simulink model "SinglePhaseGridSolarPV"  (R2025b)
settings: Solver=ode23t  StartTime=0.0  StopTime=simulation.timeSim  FixedStep=0.001  MaxStep=1/(5*solarPlant.switchFrequency)  RelTol=1e-3  AbsTol=1e-3  EnableMultiTasking=on
PreLoadFcn:
  | run('SinglePhaseGridSolarPVData');
undefined symbols (not defined in the file): closedLoop, controller, grid, protection, sensor, solarPanel, solarPlant
libraries: simulink x19, fl_lib x16, nesl_utility x16, ee_lib x8, mcbeeMathTransformLib x2, simulink_extras x1, eeSinusoidalMeasurement x1, eeRmsMeasurement x1, eePwmGenerator x1
(part 1 of 2)
CloseFcn:
  | try, close(figHandleGridconnectedSolarSinglePhase), end
  | try, clear figHandleGridconnectedSolarSinglePhase, end
  | 
  | clear simlog_SinglePhaseGridSolarPV
  | clear warnState
  | clear solarPanel grid solarPlant sensor controller protection simulation
  | clear inductorDesign closedLoop
  | clear remainingPowerPerString
  | clear simulation  MPPT  powerCircuit
  | clear incrementalConductance perturbationAndObservation
  | clear discrete average continuous
  | clear modelName X U idx t x y X U A B C D G closedLoop
  | clear npts f G magline_h phsline_h presentMPPTVariant presentInverterVariant
  | clear i inverter
  | clear xout yout tout
Description:
  | Single-Phase Grid-Connected Solar Photovoltaic System
  | 
  | %
settings Model: Creator=The MathWorks, Inc.
settings SolverCC: AlgebraicLoopSolver=TrustRegion
settings DataIOCC: MaxDataPoints=285000  SaveFormat=Array  SaveState=on  SignalLogging=off  DSMLogging=off  ReturnWorkspaceOutputs=off  SignalLoggingName=logsout_StepperMotorValidation
settings OptimizationCC: ReuseModelBlockBuffer=off  ExpressionDepthLimit=2147483647.0  InitFltsAndDblsToZero=on  LifeSpan=inf
settings DebuggingCC: UnderspecifiedInitializationDetection=Classic  MergeDetectMultiDrivingBlocksExec=none  FcnCallInpInsideContextMsg=warning  UnconnectedInputMsg=warning  UnconnectedOutputMsg=warning  UnconnectedLineMsg=warning  StateNameClashWarn=warning  PregeneratedLibrarySubsystemCodeDiagnostic=none  SFUnexpectedBacktrackingDiag=warning  SFNoUnconditionalDefaultTransitionDiag=warning  SFExecutionAtInitializationDiag=none  ArithmeticOperatorsInVariantConditions=warning
settings HardwareCC: ProdBitPerPointer=32.0  ProdBitPerSizeT=32.0  ProdBitPerPtrDiffT=32.0  ProdLargestAtomicFloat=None  ProdIntDivRoundTo=Undefined  ProdEndianess=Unspecified  ProdWordSize=32.0  ProdHWDeviceType=32-bit Generic
settings ModelReferenceCC: EnableRefExpFcnMdlSchedulingChecks=on  PropagateSignalLabelsOutOfModel=off
settings SFSimCC: SimUseLocalCustomCode=off
settings RTWCC: RTWUseLocalCustomCode=off  GPUComputeCapability=3.5  DLArmComputeVersion=19.05
settings CodeAppCC: StateflowObjectComments=on
settings GRTTargetCC: TargetLangStandard=C89/C90 (ANSI)  CombineOutputUpdateFcns=off  GRTInterface=on
settings ConfigComp: CovScope=ReferencedModels  CovMetricSettings=dw  CovSaveCumulativeToWorkspaceVar=on  CovSaveSingleToWorkspaceVar=on  CovExternalEMLEnable=off  CovSFcnEnable=off
settings SimscapeCC: SimscapeLogType=all  SimscapeLogSimulationStatistics=on  SimscapeLogName=simlog_SinglePhaseGridSolarPV  SimscapeLogLimitData=off  SimscapeLogDataHistory=285000.0

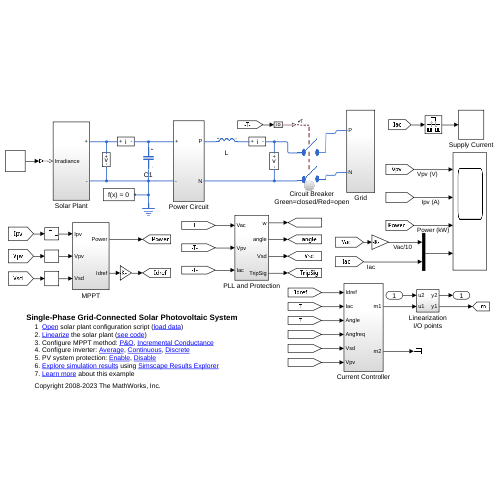
[thumbnail: Simulink's stored preview of the top-level diagram]
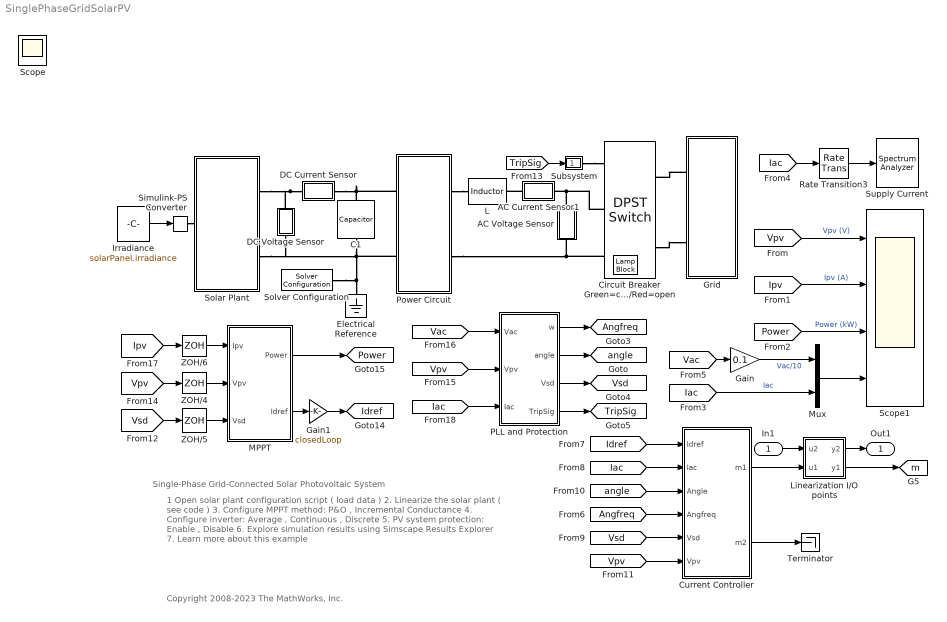
== system SinglePhaseGridSolarPV ==
  note: 1 Open solar plant configuration script ( load data )
      | 2. Linearize the solar plant ( see code )
      | 3. Configure MPPT method: P&O , Incremental Conductance
      | 4. Configure inverter: Average , Continuous , Discrete
      | 5. PV system protection: Enable , Disable
      | 6. Explore simulation results using Simscape Results Explorer
      | 7. Learn more about this example
  note: Single-Phase Grid-Connected Solar Photovoltaic System
  note: Copyright 2008-2023 The MathWorks, Inc.
  In1 : Inport
  " " : LampBlock  LabelPosition=Hide  DefaultColor=[192.0, 192.0, 192.0]
  AC Current Sensor1 : Subsystem
      mask Display: disp('i');
  AC Voltage Sensor : Subsystem
      mask Display: disp('v')
  C1 : fl_lib/Electrical/Electrical Elements/Capacitor  c=solarPlant.capacitance F  r=1e-6 Ohm  g=0 1/Ohm  i_specify=off  i_priority=High  i=0 A  i_nominal_specify=off  i_nominal_value=1  i_nominal_unit=A  v_specify=off  v_priority=High  v=0 V  v_nominal_specify=off  v_nominal_value=1  v_nominal_unit=V  vc_specify=on  vc_priority=High  vc=solarPlant.DCMPPTValue V  vc_nominal_specify=off  vc_nominal_value=1  vc_nominal_unit=V
  Circuit Breaker Green=closed/Red=open : ee_lib/Switches & Breakers/DPST Switch  R_closed=0.001 Ohm  G_open=1e-6 S  Threshold=0.5 V  Width=0 V  model_dynamics=0  t_on=1e-3 s  t_off=1e-3 s  initial_vT=0 V
      settings: InternalSimscapePortConfiguration="{\"Bottom\":[],\"Left\":[{\"id\":\"vT\",\"label\":\"vT\",\"type\":\"input\"},{\"id\":\"p1\",\"label\":\"\",\"type\":\"foundation.electrical.electrical\"},{\"id\":\"p2\",\"label\":\"\",\"type\":\"foundation.electrical.electrical\"}],\"Right\":[{\"id\":\"n1\",\"label\":\"\",\"type\":\"foundation.electrical.electrical\"},{\"id\":\"n2\",\"label\":\"\",\"type\":\"foundation.electrical.electrical\"}],\"Top\":[]}"
  Current Controller : Subsystem
  DC Current Sensor : Subsystem
      mask Display: disp('i')
  DC Voltage Sensor : Subsystem
      mask Display: disp('v');
  Electrical Reference : fl_lib/Electrical/Electrical Elements/Electrical Reference
  Gain : Gain  Gain=0.1
  Gain1 : Gain  Gain=closedLoop
  Grid : Subsystem
  Irradiance : Constant  Value=solarPanel.irradiance
  L : fl_lib/Electrical/Electrical Elements/Inductor  l=solarPlant.lineInductance H  r=solarPlant.inductorResistance Ohm  g=1e-9 1/Ohm  i_specify=off  i_priority=High  i=0 A  i_nominal_specify=off  i_nominal_value=1  i_nominal_unit=A  v_specify=off  v_priority=High  v=0 V  v_nominal_specify=off  v_nominal_value=1  v_nominal_unit=V  i_L_specify=on  i_L_priority=High  i_L=0 A  i_L_nominal_specify=off  i_L_nominal_value=1  i_L_nominal_unit=A
      settings: LogSimulationData=on
  Linearization I/O points : Subsystem
  MPPT : Subsystem
  Mux : Mux  Inputs=2
  PLL and Protection : Subsystem
  Power Circuit : Subsystem
  Rate Transition3 : RateTransition  OutPortSampleTime=1e-4
  Scope1 : Scope  NumInputPorts=4
      settings: TimeSpan=simulation.timeSim  ActiveDisplayYMinimum=-79.35501  ActiveDisplayYMaximum=714.19509
  Simulink-PS Converter : nesl_utility/Simulink-PS Converter  PhysicalDomain=network_engine_domain  SubClassName=ps_input  LeftPortType=input  RightPortType=output  PseudoPeriodic=off  Frequencies=[]  NoiseDistribution=none  NoiseParameters=[]  Unit=1  AffineConversion=off  FilteringAndDerivatives=provide  SimscapeFilterOrder=1  InputFilterTimeConstant=0.001  UdotUserProvided=0
  Solar Plant : Subsystem
  Solver Configuration : nesl_utility/Solver Configuration  PhysicalDomain=network_engine_domain  SubClassName=solver  LeftPortType=input  RightPortType=generic  Tones=[]  Harmonics=[]  SimulateNoise=off  Profile=off  UseLocalSampling=off  EnableSwitchedLinearOptims=on  FrequencyDomain=off  UseCCode=off  RelTol=0.001  AbsTol=1e-06  MinStep=1e-09  ToWorkspace=off  RevertToSquareIcSolve=off  NumHomotopyIterations=100  PhasorMode=off  PhasorModeNumHarmonics=1  ConsistencySolver=NEWTON_FTOL  IndexReductionMethod=DerivativeReplacement  DoDC=off  ResidualTolerance=1e-9  ConsistencyTolSource=GLOBAL  ConsistencyAbsTol=0.001  ConsistencyRelTol=0.001  ConsistencyTolFactor=0.001  UseLocalSolver=off  LocalSolverChoice=NE_TRAPEZOIDAL_ADVANCER  ResolveIndetEquations=on  FunctionEvalNumThread=1  LocalSolverSampleTime=1e-7  DoFixedCost=off  MaxNonlinIter=10  MaxModeIter=2  ComputeImpulses=off  ImpulseIterations=2  LinearAlgebra=auto  LinearAlgebraNumThread=0  EquationFormulation=NE_TIME_EF  DelaysMemoryBudget=1024  AutomaticFiltering=on  FilteringTimeConstant=0.001  PartitionStorageMethod=AS_NEEDED  PartitionMemoryBudget=1024  PartitionMethod=FAST  MultibodyUseLocalSolver=off  MultibodyLocalSolverChoice=ODE1  MultibodyLocalSolverSampleTime=0.001
  Subsystem : Subsystem
  Supply Current : SpectrumAnalyzer  WindowPosition=[886 344 803 532]  SpectrumType=RMS  Method=Welch  PlotAsTwoSidedSpectrum=off  FrequencyScale=Log  AxesScaling=Manual  RBWSource=Property  RBW=9  Span=5000  CenterFrequency=2500  StartFrequency=0  OverlapPercent=90  AveragingMethod=Running  SpectrumUnits=Vrms  YLimits=[-2.1499375144550283423,19.349555712689415543]  ColorLimits=[0.0061790664803535039207,16.888204283875005274]  AllowFFTLengthLessThanSamplesPerUpdate=on
      settings: OpenAtSimulationStart=off
  Terminator : Terminator
  ZOH/4 : ZeroOrderHold  SampleTime=solarPlant.timeMPPT
  ZOH/5 : ZeroOrderHold  SampleTime=solarPlant.timeMPPT
  ZOH/6 : ZeroOrderHold  SampleTime=solarPlant.timeMPPT
  Out1 : Outport  VectorParamsAs1DForOutWhenUnconnected=off
  Scope : Scope
      settings: ActiveDisplayYMinimum=-0.0002  ActiveDisplayYMaximum=0.0018
  tag scope: Angfreq=global, Idref=global, Power=global, TripSig=global, Vsd=global, angle=global, m=global
  wires:
  Mux/1 -> Scope1/4
  Irradiance/1 -> Simulink-PS Converter/1
  [Vsd] -> ZOH/5/1
  [Vpv] -> ZOH/4/1
  [Iac] -> Current Controller/2(Iac)
  Current Controller/1(m1) -> Linearization I/O points/2(u1)
  [Vac] -> Gain/1
  PLL and Protection/4(TripSig) -> [TripSig]
  Rate Transition3/1 -> Supply Current/1
  PLL and Protection/2(angle) -> [angle]
  [TripSig] -> Subsystem/1(i)
  Linearization I/O points/1(y2) -> Out1/1
  [Iac] -> PLL and Protection/3(Iac)
  ZOH/5/1 -> MPPT/3(Vsd)
  PLL and Protection/3(Vsd) -> [Vsd]
  [Vac] -> PLL and Protection/1(Vac)
  [Ipv] -> Scope1/2  "Ipv (A)"
  Linearization I/O points/2(y1) -> [m]
  [Vsd] -> Current Controller/5(Vsd)
  Current Controller/2(m2) -> Terminator/1
  PLL and Protection/1(w) -> [Angfreq]
  [Angfreq] -> Current Controller/4(Angfreq)
  [Ipv] -> ZOH/6/1
  [Vpv] -> Scope1/1  "Vpv (V)"
  [Idref] -> Current Controller/1(Idref)
  MPPT/2(Idref) -> Gain1/1
  Gain1/1 -> [Idref]
  [Vpv] -> PLL and Protection/2(Vpv)
  [Vpv] -> Current Controller/6(Vpv)
  In1/1 -> Linearization I/O points/1(u2)
  [Iac] -> Mux/2  "Iac"
  [Power] -> Scope1/3  "Power (kW)"
  [angle] -> Current Controller/3(Angle)
  ZOH/4/1 -> MPPT/2(Vpv)
  ZOH/6/1 -> MPPT/1(Ipv)
  Gain/1 -> Mux/1  "Vac/10"
  [Iac] -> Rate Transition3/1
  MPPT/1(Power) -> [Power]
  connections:
  Power Circuit/LConn2 -- Electrical Reference/LConn1 -- Solver Configuration/RConn1 -- C1/RConn1 -- Solar Plant/RConn2 -- DC Voltage Sensor/LConn1
  Circuit Breaker Green=closed/Red=open/LConn3 -- Power Circuit/RConn2 -- AC Voltage Sensor/LConn1
  DC Current Sensor/RConn1 -- Solar Plant/RConn1 -- DC Voltage Sensor/RConn1
  AC Current Sensor1/LConn1 -- AC Voltage Sensor/RConn1 -- Circuit Breaker Green=closed/Red=open/LConn2
  Power Circuit/LConn1 -- DC Current Sensor/LConn1 -- C1/LConn1
  Grid/LConn1 -- Circuit Breaker Green=closed/Red=open/RConn1
  Circuit Breaker Green=closed/Red=open/RConn2 -- Grid/LConn2
  AC Current Sensor1/RConn1 -- L/RConn1
  Subsystem/RConn1 -- Circuit Breaker Green=closed/Red=open/LConn1
  Simulink-PS Converter/RConn1 -- Solar Plant/LConn1
  Power Circuit/RConn1 -- L/LConn1

== system SinglePhaseGridSolarPV/AC Current Sensor1 ==
  Current Sensor : fl_lib/Electrical/Electrical Sensors/Current Sensor
  PS-Simulink Converter : nesl_utility/PS-Simulink Converter  PhysicalDomain=network_engine_domain  SubClassName=ps_output  LeftPortType=input  RightPortType=output  PseudoPeriodic=off  Frequencies=[]  VectorFormat=1-D array  Unit=1  AffineConversion=off
  Sensor dynamics : TransferFcn  Numerator=1  Denominator=[1/sensor.samplingFreq 1]
  - : PMIOPort  Side=Left
  + : PMIOPort  Port=2  Side=Right
  tag scope: Iac=global
  wires:
  PS-Simulink Converter/1 -> Sensor dynamics/1
  Sensor dynamics/1 -> [Iac]
  connections:
  Current Sensor/RConn1 -- PS-Simulink Converter/LConn1
  +/RConn1 -- Current Sensor/LConn1
  Current Sensor/RConn2 -- -/RConn1

== system SinglePhaseGridSolarPV/AC Voltage Sensor ==
  PS-Simulink Converter : nesl_utility/PS-Simulink Converter  PhysicalDomain=network_engine_domain  SubClassName=ps_output  LeftPortType=input  RightPortType=output  PseudoPeriodic=off  Frequencies=[]  VectorFormat=1-D array  Unit=1  AffineConversion=off
  Sensor dynamics : TransferFcn  Numerator=1  Denominator=[1/sensor.samplingFreq 1]
  Voltage Sensor : fl_lib/Electrical/Electrical Sensors/Voltage Sensor
  - : PMIOPort  Side=Left
  + : PMIOPort  Port=2  Side=Right
  tag scope: Vac=global
  wires:
  PS-Simulink Converter/1 -> Sensor dynamics/1
  Sensor dynamics/1 -> [Vac]
  connections:
  Voltage Sensor/RConn2 -- -/RConn1
  Voltage Sensor/RConn1 -- PS-Simulink Converter/LConn1
  Voltage Sensor/LConn1 -- +/RConn1

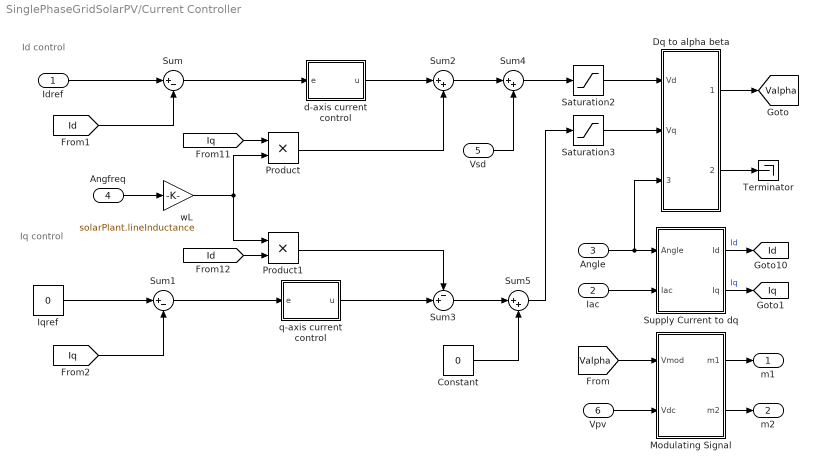
== system SinglePhaseGridSolarPV/Current Controller ==
  note: Iq control
  note: Id control
  Idref : Inport
  Iac : Inport  Port=2
  Angle : Inport  Port=3
  Angfreq : Inport  Port=4
  Vsd : Inport  Port=5
  Vpv : Inport  Port=6
  Constant : Constant  Value=0
  Dq to alpha beta : Subsystem
  Iqref : Constant  Value=0
  Modulating Signal : Subsystem
  Product : Product
  Product1 : Product
  Saturation2 : Saturate  UpperLimit=controller.currentVoltMax*1.5  LowerLimit=-1*controller.currentVoltMax*1.5
  Saturation3 : Saturate  UpperLimit=controller.currentVoltMax*1.5  LowerLimit=-1*controller.currentVoltMax*1.5
  Sum : Sum  Inputs=|+-
  Sum1 : Sum  Inputs=|+-
  Sum2 : Sum  Inputs=|++
  Sum3 : Sum  Inputs=-+|
  Sum4 : Sum  Inputs=|++
  Sum5 : Sum  Inputs=|++
  Supply Current to dq : Subsystem
  Terminator : Terminator
  d-axis current control : Subsystem
  q-axis current control : Subsystem
  wL : Gain  Gain=solarPlant.lineInductance
  m1 : Outport  VectorParamsAs1DForOutWhenUnconnected=off
  m2 : Outport  Port=2  VectorParamsAs1DForOutWhenUnconnected=off
  tag scope: Id=global, Iq=global, Valpha=global
  wires:
  Sum1/1 -> q-axis current control/1(e)
  wL/1 -> Product/2, Product1/1
  [Id] -> Product1/2
  [Iq] -> Product/1
  Product1/1 -> Sum3/1
  Product/1 -> Sum2/2
  Sum3/1 -> Sum5/1
  Sum2/1 -> Sum4/1
  Modulating Signal/1(m1) -> m1/1
  Modulating Signal/2(m2) -> m2/1
  Sum4/1 -> Saturation2/1
  Sum5/1 -> Saturation3/1
  Angfreq/1 -> wL/1
  Constant/1 -> Sum5/2
  Angle/1 -> Dq to alpha beta/3(angle), Supply Current to dq/1(Angle)
  [Valpha] -> Modulating Signal/1(Vmod)
  Vpv/1 -> Modulating Signal/2(Vdc)
  Sum/1 -> d-axis current control/1(e)
  [Id] -> Sum/2
  d-axis current control/1(u) -> Sum2/1
  q-axis current control/1(u) -> Sum3/2
  Supply Current to dq/1(Id) -> [Id]  "Id"
  Supply Current to dq/2(Iq) -> [Iq]  "Iq"
  Iac/1 -> Supply Current to dq/2(Iac)
  Saturation2/1 -> Dq to alpha beta/1("Vd ")
  Saturation3/1 -> Dq to alpha beta/2(Vq)
  Vsd/1 -> Sum4/2
  Dq to alpha beta/1(Valpha) -> [Valpha]
  Dq to alpha beta/2(Vbeta) -> Terminator/1
  Iqref/1 -> Sum1/1
  [Iq] -> Sum1/2
  Idref/1 -> Sum/1

== system SinglePhaseGridSolarPV/DC Current Sensor ==
  Current Sensor : fl_lib/Electrical/Electrical Sensors/Current Sensor
      settings: LogSimulationData=on
  PS-Simulink Converter : nesl_utility/PS-Simulink Converter  PhysicalDomain=network_engine_domain  SubClassName=ps_output  LeftPortType=input  RightPortType=output  PseudoPeriodic=off  Frequencies=[]  VectorFormat=1-D array  Unit=1  AffineConversion=off
  Sensor dynamics : TransferFcn  Numerator=1  Denominator=[1/sensor.samplingFreq 1]
  - : PMIOPort  Side=Left
  + : PMIOPort  Port=2  Side=Right
  tag scope: Ipv=global
  wires:
  PS-Simulink Converter/1 -> Sensor dynamics/1
  Sensor dynamics/1 -> [Ipv]
  connections:
  Current Sensor/RConn2 -- -/RConn1
  +/RConn1 -- Current Sensor/LConn1
  Current Sensor/RConn1 -- PS-Simulink Converter/LConn1

== system SinglePhaseGridSolarPV/DC Voltage Sensor ==
  PS-Simulink Converter : nesl_utility/PS-Simulink Converter  PhysicalDomain=network_engine_domain  SubClassName=ps_output  LeftPortType=input  RightPortType=output  PseudoPeriodic=off  Frequencies=[]  VectorFormat=1-D array  Unit=1  AffineConversion=off
  Sensor dynamics : TransferFcn  Numerator=1  Denominator=[1/sensor.samplingFreq 1]
  Voltage Sensor : fl_lib/Electrical/Electrical Sensors/Voltage Sensor
      settings: LogSimulationData=on
  - : PMIOPort  Side=Left
  + : PMIOPort  Port=2  Side=Right
  tag scope: Vpv=global
  wires:
  PS-Simulink Converter/1 -> Sensor dynamics/1
  Sensor dynamics/1 -> [Vpv]
  connections:
  Voltage Sensor/LConn1 -- +/RConn1
  Voltage Sensor/RConn1 -- PS-Simulink Converter/LConn1
  Voltage Sensor/RConn2 -- -/RConn1

== system SinglePhaseGridSolarPV/Grid ==
  Controlled Voltage Source : fl_lib/Electrical/Electrical Sources/Controlled Voltage Source
  Grid Supply : Sin  Amplitude=grid.actualVoltage*sqrt(2)  Frequency=grid.frequency*2*pi  SampleTime=0
  Product : Product
  Simulink-PS Converter : nesl_utility/Simulink-PS Converter  PhysicalDomain=network_engine_domain  SubClassName=ps_input  LeftPortType=input  RightPortType=output  PseudoPeriodic=off  Frequencies=[]  NoiseDistribution=none  NoiseParameters=[]  Unit=1  AffineConversion=off  FilteringAndDerivatives=provide  SimscapeFilterOrder=1  InputFilterTimeConstant=0.001  UdotUserProvided=0
  Voltage Distrubance : Step  Time=10  Before=1  After=1.05  SampleTime=0
  P : PMIOPort  Side=Left
  N : PMIOPort  Port=2  Side=Left
  wires:
  Grid Supply/1 -> Product/2
  Product/1 -> Simulink-PS Converter/1
  Voltage Distrubance/1 -> Product/1
  connections:
  P/RConn1 -- Controlled Voltage Source/LConn1
  N/RConn1 -- Controlled Voltage Source/RConn2
  Simulink-PS Converter/RConn1 -- Controlled Voltage Source/RConn1

== system SinglePhaseGridSolarPV/Linearization I//O points ==
  u2 : Inport
  u1 : Inport  Port=2
  "Set to 1 for closed-loop operation, and set to 0 when linearizing" : Gain  Gain=closedLoop  SaturateOnIntegerOverflow=on  OutDataTypeStr=Inherit: Same as input  ParamDataTypeStr=Inherit: Same as input
  Sum1 : Sum  Inputs=++|  InputSameDT=on  SaturateOnIntegerOverflow=on  OutDataTypeStr=Inherit: Same as first input
  y2 : Outport  VectorParamsAs1DForOutWhenUnconnected=off
  y1 : Outport  Port=2  VectorParamsAs1DForOutWhenUnconnected=off
  wires:
  Sum1/1 -> y1/1
  u2/1 -> Sum1/1
  "Set to 1 for closed-loop operation, and set to 0 when linearizing"/1 -> Sum1/2
  u1/1 -> y2/1, "Set to 1 for closed-loop operation, and set to 0 when linearizing"/1

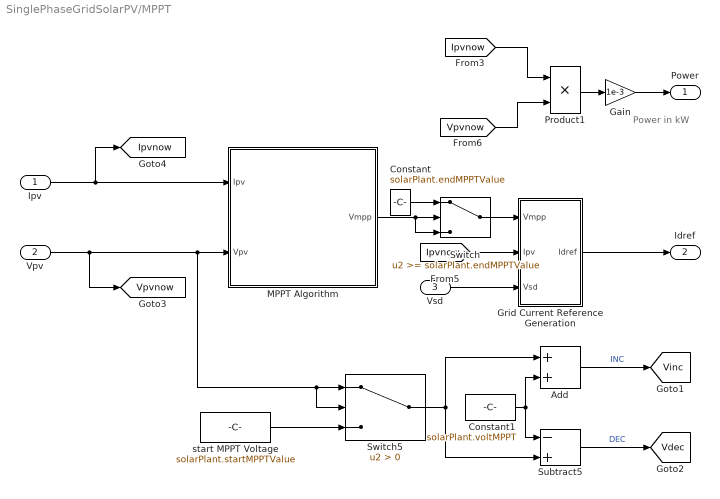
== system SinglePhaseGridSolarPV/MPPT ==
  note: Power in kW
  Ipv : Inport
  Vpv : Inport  Port=2
  Vsd : Inport  Port=3
  Add : Sum
  Constant : Constant  Value=solarPlant.endMPPTValue
  Constant1 : Constant  Value=solarPlant.voltMPPT
  Gain : Gain  Gain=1e-3
  Grid Current Reference Generation : Subsystem
  MPPT Algorithm : Subsystem  Variant=on
  Product1 : Product
  Subtract5 : Sum  Inputs=-+
  Switch : Switch  Threshold=solarPlant.endMPPTValue  SaturateOnIntegerOverflow=off  InputSameDT=off
  Switch5 : Switch  Criteria=u2 > Threshold  SaturateOnIntegerOverflow=off  InputSameDT=off
  start MPPT Voltage : Constant  Value=solarPlant.startMPPTValue
  Power : Outport  VectorParamsAs1DForOutWhenUnconnected=off
  Idref : Outport  Port=2  VectorParamsAs1DForOutWhenUnconnected=off
  tag scope: Ipvnow=global, Vdec=global, Vinc=global, Vpvnow=global
  wires:
  Switch5/1 -> Add/1, Subtract5/2
  Add/1 -> [Vinc]  "INC"
  start MPPT Voltage/1 -> Switch5/3
  Vpv/1 -> [Vpvnow], Switch5/2, Switch5/1, MPPT Algorithm/2(Vpv)
  Constant1/1 -> Add/2, Subtract5/1
  [Ipvnow] -> Grid Current Reference Generation/2(Ipv)
  Grid Current Reference Generation/1(Idref) -> Idref/1
  [Vpvnow] -> Product1/2
  [Ipvnow] -> Product1/1
  Product1/1 -> Gain/1
  Vsd/1 -> Grid Current Reference Generation/3(Vsd)
  Subtract5/1 -> [Vdec]  "DEC"
  Ipv/1 -> [Ipvnow], MPPT Algorithm/1(Ipv)
  Gain/1 -> Power/1
  Switch/1 -> Grid Current Reference Generation/1(Vmpp)
  MPPT Algorithm/1(Vmpp) -> Switch/3, Switch/2
  Constant/1 -> Switch/1

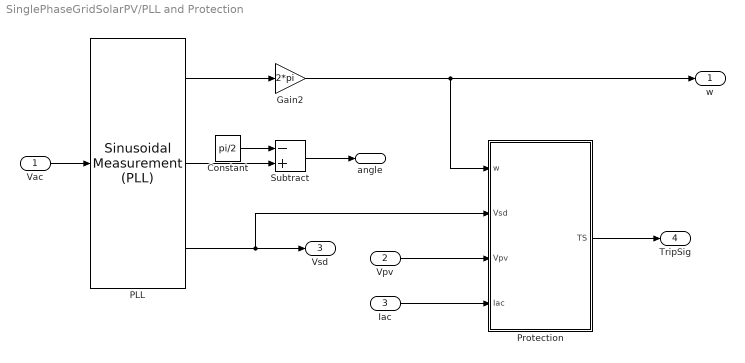
== system SinglePhaseGridSolarPV/PLL and Protection ==
  Vac : Inport
  Vpv : Inport  Port=2
  Iac : Inport  Port=3
  Constant : Constant  Value=pi/2
  Gain2 : Gain  Gain=2*pi
  PLL : eeSinusoidalMeasurement/Sinusoidal Measurement (PLL)  Ki_PD=600  Kp_LF=10  Ki_LF=200  F0=grid.frequency  Theta0=0  Mag0=grid.actualVoltage*sqrt(2)  Ts=0
  Protection : Subsystem
  Subtract : Sum  Inputs=-+
  w : Outport  VectorParamsAs1DForOutWhenUnconnected=off
  angle : Outport  Port=2  VectorParamsAs1DForOutWhenUnconnected=off
  Vsd : Outport  Port=3  VectorParamsAs1DForOutWhenUnconnected=off
  TripSig : Outport  Port=4  VectorParamsAs1DForOutWhenUnconnected=off
  wires:
  PLL/3 -> Vsd/1, Protection/2(Vsd)
  Gain2/1 -> Protection/1(w), w/1
  PLL/1 -> Gain2/1
  Vac/1 -> PLL/1
  Protection/1(TS) -> TripSig/1
  Vpv/1 -> Protection/3(Vpv)
  Iac/1 -> Protection/4(Iac)
  Subtract/1 -> angle/1
  PLL/2 -> Subtract/2
  Constant/1 -> Subtract/1

== system SinglePhaseGridSolarPV/Power Circuit ==
  Power Circuit : Subsystem  Variant=on  VariantControl=Variant1
  + : PMIOPort  Side=Left
  P : PMIOPort  Port=2  Side=Right
  N : PMIOPort  Port=3  Side=Right
  - : PMIOPort  Port=4  Side=Left
  wires:
  [m] -> Power Circuit/1(m)
  [TripSig] -> Power Circuit/2(TripSig)
  connections:
  +/RConn1 -- Power Circuit/LConn1
  -/RConn1 -- Power Circuit/LConn2
  P/RConn1 -- Power Circuit/RConn1
  N/RConn1 -- Power Circuit/RConn2

== system SinglePhaseGridSolarPV/Solar Plant ==
  Current-Controlled Current Source- Scale panel current to Np parallel strings : fl_lib/Electrical/Electrical Sources/Current-Controlled Current Source  K=-1*(solarPlant.numParallelPanel-1)  i1_specify=off  i1_priority=None  i1=0 A  i1_nominal_specify=off  i1_nominal_value=1  i1_nominal_unit=A  i2_specify=off  i2_priority=None  i2=0 A  i2_nominal_specify=off  i2_nominal_value=1  i2_nominal_unit=A
      settings: InternalSimscapePortConfiguration="{\"Bottom\":[],\"Left\":[{\"id\":\"p1\",\"label\":\"+\",\"type\":\"foundation.electrical.electrical\"},{\"id\":\"head\",\"label\":\"\",\"type\":\"foundation.electrical.electrical\"}],\"Right\":[{\"id\":\"n1\",\"label\":\"-\",\"type\":\"foundation.electrical.electrical\"},{\"id\":\"tail\",\"label\":\"\",\"type\":\"foundation.electrical.electrical\"}],\"Top\":[]}"
  Solar Panel : Subsystem  mask(Solar Panel){}
      mask help: Models a solar panel using a parallel-connected sting of solar cells. The solar cell strings are modeled using a single Solar Cell block from the Simscape(TM) Electrical(TM) Sources library.
      mask Display: image('SolarPanelValidationIcon.jpg')
  Voltage-Controlled Voltage Source - Scale panel voltage to Ns series panel : fl_lib/Electrical/Electrical Sources/Voltage-Controlled Voltage Source  K=-1*(solarPlant.numSeriesPanel-1)  v1_specify=off  v1_priority=None  v1=0 V  v1_nominal_specify=off  v1_nominal_value=1  v1_nominal_unit=V  v2_specify=off  v2_priority=None  v2=0 V  v2_nominal_specify=off  v2_nominal_value=1  v2_nominal_unit=V
      settings: InternalSimscapePortConfiguration="{\"Bottom\":[],\"Left\":[{\"id\":\"p1\",\"label\":\"+\",\"type\":\"foundation.electrical.electrical\"},{\"id\":\"p2\",\"label\":\"+\",\"type\":\"foundation.electrical.electrical\"}],\"Right\":[{\"id\":\"n1\",\"label\":\"-\",\"type\":\"foundation.electrical.electrical\"},{\"id\":\"n2\",\"label\":\"-\",\"type\":\"foundation.electrical.electrical\"}],\"Top\":[]}"
  + : PMIOPort  Side=Right
  Irradiance : PMIOPort  Port=2  Side=Left
  - : PMIOPort  Port=3  Side=Right
  connections:
  Voltage-Controlled Voltage Source - Scale panel voltage to Ns series panel/RConn2 -- Voltage-Controlled Voltage Source - Scale panel voltage to Ns series panel/RConn1 -- Solar Panel/RConn1
  Voltage-Controlled Voltage Source - Scale panel voltage to Ns series panel/LConn1 -- Current-Controlled Current Source- Scale panel current to Np parallel strings/LConn2 -- -/RConn1 -- Solar Panel/RConn2
  Current-Controlled Current Source- Scale panel current to Np parallel strings/RConn1 -- Current-Controlled Current Source- Scale panel current to Np parallel strings/RConn2 -- +/RConn1
  Current-Controlled Current Source- Scale panel current to Np parallel strings/LConn1 -- Voltage-Controlled Voltage Source - Scale panel voltage to Ns series panel/LConn2
  Solar Panel/LConn1 -- Irradiance/RConn1

== system SinglePhaseGridSolarPV/Subsystem ==
  i : Inport
  Data Type Conversion : DataTypeConversion  SaturateOnIntegerOverflow=off  RndMeth=Floor
  NOT : Logic  Operator=NOT  IconShape=distinctive  AllPortsSameDT=off  OutDataTypeStr=boolean
  Simulink-PS Converter : nesl_utility/Simulink-PS Converter  PhysicalDomain=network_engine_domain  SubClassName=ps_input  LeftPortType=input  RightPortType=output  PseudoPeriodic=off  Frequencies=[]  NoiseDistribution=none  NoiseParameters=[]  Unit=1  AffineConversion=off  FilteringAndDerivatives=provide  SimscapeFilterOrder=1  InputFilterTimeConstant=0.001  UdotUserProvided=0
  o : PMIOPort  Side=Right
  wires:
  NOT/1 -> Data Type Conversion/1
  i/1 -> NOT/1
  Data Type Conversion/1 -> Simulink-PS Converter/1
  connections:
  Simulink-PS Converter/RConn1 -- o/RConn1

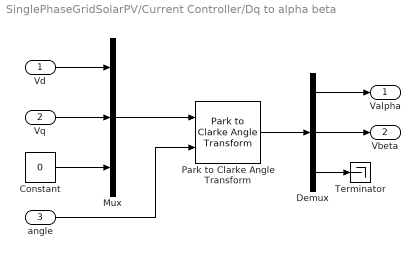
== system SinglePhaseGridSolarPV/Current Controller/Dq to alpha beta ==
  "Vd " : Inport
  Vq : Inport  Port=2
  angle : Inport  Port=3
  Constant : Constant  Value=0
  Demux : Demux  Outputs=3
  Mux : Mux  Inputs=3
  Park to Clarke Angle Transform : mcbeeMathTransformLib/Park to Clarke Angle Transform  AxisAlignment=D-axis  UseWithEmbedded=off  PhaseInput=Two inputs  ThetaInput=Sine and Cosine electrical position  AngleInput=Per-unit  N_points=1024
      settings: LibrarySourceBlock=|
      | eeTransforms/Park to Clarke
      | Angle Transform
  Terminator : Terminator
  Valpha : Outport  VectorParamsAs1DForOutWhenUnconnected=off
  Vbeta : Outport  Port=2  VectorParamsAs1DForOutWhenUnconnected=off
  wires:
  "Vd "/1 -> Mux/1
  Vq/1 -> Mux/2
  Constant/1 -> Mux/3
  Mux/1 -> Park to Clarke Angle Transform/1
  angle/1 -> Park to Clarke Angle Transform/2
  Park to Clarke Angle Transform/1 -> Demux/1
  Demux/1 -> Valpha/1
  Demux/2 -> Vbeta/1
  Demux/3 -> Terminator/1

== system SinglePhaseGridSolarPV/Current Controller/Modulating Signal ==
  Vmod : Inport
  Vdc : Inport  Port=2
  Gain : Gain  Gain=-1
  Normalize by DC voltage and disable if DC volts too low : Subsystem
  "[-1,1]" : Saturate  UpperLimit=1  LowerLimit=-1
  m1 : Outport  VectorParamsAs1DForOutWhenUnconnected=off
  m2 : Outport  Port=2  VectorParamsAs1DForOutWhenUnconnected=off
  wires:
  Normalize by DC voltage and disable if DC volts too low/1(y) -> "[-1,1]"/1
  Vdc/1 -> Normalize by DC voltage and disable if DC volts too low/2(v_dc)
  Vmod/1 -> Normalize by DC voltage and disable if DC volts too low/1(u)
  "[-1,1]"/1 -> m1/1, Gain/1
  Gain/1 -> m2/1

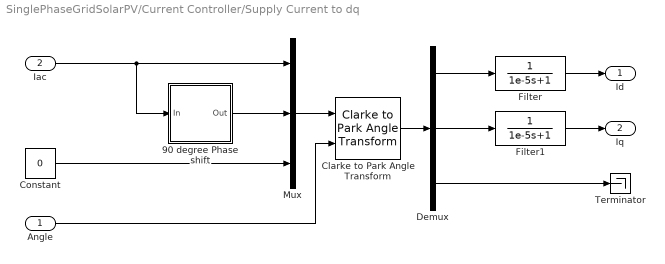
== system SinglePhaseGridSolarPV/Current Controller/Supply Current to dq ==
  Angle : Inport
  Iac : Inport  Port=2
  90 degree Phase shift : Subsystem
  Clarke to Park Angle Transform : mcbeeMathTransformLib/Clarke to Park Angle Transform  AxisAlignment=D-axis  UseWithEmbedded=off  PhaseInput=Two inputs  ThetaInput=Sine and Cosine electrical position  AngleInput=Per-unit  N_points=1024
      settings: LibrarySourceBlock=|
      | eeTransforms/Clarke to Park
      | Angle Transform
  Constant : Constant  Value=0
  Demux : Demux  Outputs=3
  Filter : TransferFcn  Denominator=[1e-5 1]
  Filter1 : TransferFcn  Denominator=[1e-5 1]
  Mux : Mux  Inputs=3
  Terminator : Terminator
  Id : Outport  VectorParamsAs1DForOutWhenUnconnected=off
  Iq : Outport  Port=2  VectorParamsAs1DForOutWhenUnconnected=off
  wires:
  Constant/1 -> Mux/3
  Mux/1 -> Clarke to Park Angle Transform/1
  Angle/1 -> Clarke to Park Angle Transform/2
  Demux/1 -> Filter/1
  Clarke to Park Angle Transform/1 -> Demux/1
  Demux/3 -> Terminator/1
  Filter/1 -> Id/1
  Iac/1 -> 90 degree Phase shift/1(In), Mux/1
  90 degree Phase shift/1(Out) -> Mux/2
  Filter1/1 -> Iq/1
  Demux/2 -> Filter1/1

== system SinglePhaseGridSolarPV/Current Controller/d-axis current control ==
  e : Inport
  Integrator : Integrator  LimitOutput=on  UpperSaturationLimit=controller.currentVoltMax  LowerSaturationLimit=-controller.currentVoltMax
  Ki : Gain  Gain=1/controller.currentPole
  Kp : Gain  Gain=controller.currentGain
  Saturation : Saturate  UpperLimit=controller.currentVoltMax  LowerLimit=-1*controller.currentVoltMax
  Sum7 : Sum  Inputs=|++
  u : Outport  VectorParamsAs1DForOutWhenUnconnected=off
  wires:
  Integrator/1 -> Sum7/2
  Saturation/1 -> u/1
  Sum7/1 -> Saturation/1
  e/1 -> Kp/1
  Kp/1 -> Ki/1, Sum7/1
  Ki/1 -> Integrator/1

== system SinglePhaseGridSolarPV/Current Controller/q-axis current control ==
  e : Inport
  Integrator : Integrator  LimitOutput=on  UpperSaturationLimit=controller.currentVoltMax  LowerSaturationLimit=-controller.currentVoltMax
  Ki : Gain  Gain=1/controller.currentPole
  Kp : Gain  Gain=controller.currentGain
  Saturation : Saturate  UpperLimit=controller.currentVoltMax  LowerLimit=-1*controller.currentVoltMax
  Sum7 : Sum  Inputs=|++
  u : Outport  VectorParamsAs1DForOutWhenUnconnected=off
  wires:
  Ki/1 -> Integrator/1
  Kp/1 -> Sum7/1, Ki/1
  e/1 -> Kp/1
  Sum7/1 -> Saturation/1
  Saturation/1 -> u/1
  Integrator/1 -> Sum7/2

== system SinglePhaseGridSolarPV/MPPT/Grid Current Reference Generation ==
  Vmpp : Inport
  Ipv : Inport  Port=2
  Vsd : Inport  Port=3
  Divide : Product  Inputs=*/
  Gain : Gain  Gain=2
  Product : Product
  Switch1 : Switch  Criteria=u2 > Threshold  Threshold=sqrt(2)*grid.actualVoltage*0.5  SaturateOnIntegerOverflow=off  InputSameDT=off
  Transfer Fcn (with initial outputs) : simulink_extras/Additional Linear/Transfer Fcn (with initial outputs)  N=[1]  D="[solarPlant.timeMPPT*70  1]"  Y0=solarPlant.initialIsdCurrent  U0=solarPlant.initialIsdCurrent
  Vsd Default : Constant  Value=sqrt(2)*grid.actualVoltage
  Idref : Outport  VectorParamsAs1DForOutWhenUnconnected=off
  wires:
  Divide/1 -> Gain/1
  Product/1 -> Divide/1
  Switch1/1 -> Divide/2
  Gain/1 -> Transfer Fcn (with initial outputs)/1
  Vmpp/1 -> Product/1
  Vsd/1 -> Switch1/2, Switch1/1
  Vsd Default/1 -> Switch1/3
  Ipv/1 -> Product/2
  Transfer Fcn (with initial outputs)/1 -> Idref/1

== system SinglePhaseGridSolarPV/MPPT/MPPT Algorithm ==
  Ipv : Inport
  Vpv : Inport  Port=2
  IncrementalConductance : Subsystem  VariantControl=incrementalConductance
  PerturbationAndObsrvation : Subsystem  VariantControl=perturbationAndObservation
  Vmpp : Outport  VectorParamsAs1DForOutWhenUnconnected=off

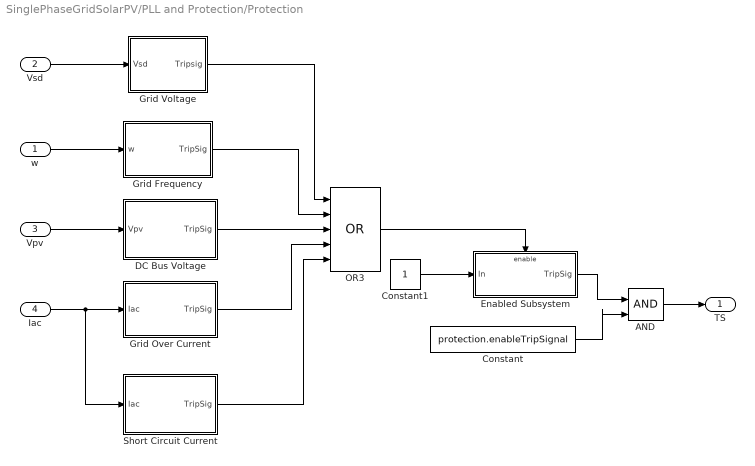
== system SinglePhaseGridSolarPV/PLL and Protection/Protection ==
  w : Inport
  Vsd : Inport  Port=2
  Vpv : Inport  Port=3
  Iac : Inport  Port=4
  AND : Logic  IconShape=distinctive  AllPortsSameDT=off  OutDataTypeStr=boolean
  Constant : Constant  Value=protection.enableTripSignal
  Constant1 : Constant
  DC Bus Voltage : Subsystem
  Enabled Subsystem : Subsystem  TreatAsAtomicUnit=on
  Grid Frequency : Subsystem
  Grid Over Current : Subsystem
  Grid Voltage : Subsystem
  OR3 : Logic  Operator=OR  Inputs=5  IconShape=distinctive  AllPortsSameDT=off  OutDataTypeStr=boolean
  Short Circuit Current : Subsystem
  TS : Outport  VectorParamsAs1DForOutWhenUnconnected=off
  wires:
  Constant1/1 -> Enabled Subsystem/1(In)
  Iac/1 -> Grid Over Current/1(Iac), Short Circuit Current/1(Iac)
  OR3/1 -> Enabled Subsystem/Enable
  Vsd/1 -> Grid Voltage/1(Vsd)
  Grid Voltage/1(Tripsig) -> OR3/1
  w/1 -> Grid Frequency/1(w)
  Grid Frequency/1(TripSig) -> OR3/2
  Vpv/1 -> DC Bus Voltage/1(Vpv)
  DC Bus Voltage/1(TripSig) -> OR3/3
  Grid Over Current/1(TripSig) -> OR3/4
  Short Circuit Current/1(TripSig) -> OR3/5
  Enabled Subsystem/1(TripSig) -> AND/1
  Constant/1 -> AND/2
  AND/1 -> TS/1

== system SinglePhaseGridSolarPV/Power Circuit/Power Circuit ==
  m : Inport
  TripSig : Inport  Port=2
  Average : Subsystem  VariantControl=average
  Continuous : Subsystem  VariantControl=continuous
  Discrete : Subsystem  VariantControl=discrete
  P : PMIOPort  Side=Right
  + : PMIOPort  Port=2  Side=Left
  - : PMIOPort  Port=3  Side=Left
  N : PMIOPort  Port=4  Side=Right

== system SinglePhaseGridSolarPV/Solar Plant/Solar Panel ==
  Current-Controlled Current Source : fl_lib/Electrical/Electrical Sources/Current-Controlled Current Source  K=-1*(solarPanel.numParallelCell-1)  i1_specify=off  i1_priority=None  i1=0 A  i1_nominal_specify=off  i1_nominal_value=1  i1_nominal_unit=A  i2_specify=off  i2_priority=None  i2=0 A  i2_nominal_specify=off  i2_nominal_value=1  i2_nominal_unit=A
      settings: InternalSimscapePortConfiguration="{\"Bottom\":[],\"Left\":[{\"id\":\"p1\",\"label\":\"+\",\"type\":\"foundation.electrical.electrical\"},{\"id\":\"head\",\"label\":\"\",\"type\":\"foundation.electrical.electrical\"}],\"Right\":[{\"id\":\"n1\",\"label\":\"-\",\"type\":\"foundation.electrical.electrical\"},{\"id\":\"tail\",\"label\":\"\",\"type\":\"foundation.electrical.electrical\"}],\"Top\":[]}"
  Solar Cell : ee_lib/Sources/Solar Cell  prm=1  Isc=solarPanel.shortCircuitCurrentPV/solarPanel.numParallelCell A  Voc=solarPanel.openCircuitVoltagePV/solarPanel.numSeriesCell V  Is=1e-6 A  Is2=0 A  Iph=7.34 A  Ir0=solarPanel.irradianceMeasurement W/m^2  ec=solarPanel.qualityFactor  N2=2  Rs=solarPanel.seriesResistance Ohm  Rp=inf Ohm  N_series=solarPanel.numSeriesCell-1  N_parallel=1  TIPH1=solarPanel.currentTemperatureCoeff 1/K  EG=1.11 eV  TXIS1=solarPanel.temperatureExponent  TXIS2=3  TRS1=0  TRP1=0  Tmeas=solarPanel.temperatureMeasurement degC  TFIXED=solarPanel.temperature degC  thermal_mass=100 J/K  initial_temperature=25 degC
  Ir : PMIOPort  Side=Left
  + : PMIOPort  Port=2  Side=Right
  - : PMIOPort  Port=3  Side=Right
  connections:
  Current-Controlled Current Source/LConn2 -- -/RConn1 -- Solar Cell/RConn1
  Ir/RConn1 -- Solar Cell/LConn1
  Current-Controlled Current Source/LConn1 -- Solar Cell/LConn2
  Current-Controlled Current Source/RConn1 -- Current-Controlled Current Source/RConn2 -- +/RConn1

== system SinglePhaseGridSolarPV/Current Controller/Modulating Signal/Normalize by DC voltage and disable if DC volts too low ==
  u : Inport
  v_dc : Inport  Port=2
  Min DC voltage : Constant  Value=0.5*solarPlant.startMPPTValue
  Product1 : Product  Inputs=*/  InputSameDT=on  SaturateOnIntegerOverflow=on  OutDataTypeStr=Inherit: Same as first input
  Switch1 : Switch  Threshold=0.5*solarPlant.maxPowerVoltage  SaturateOnIntegerOverflow=off
  y : Outport  VectorParamsAs1DForOutWhenUnconnected=off
  wires:
  Min DC voltage/1 -> Switch1/3
  Switch1/1 -> Product1/2
  v_dc/1 -> Switch1/2, Switch1/1
  u/1 -> Product1/1
  Product1/1 -> y/1

== system SinglePhaseGridSolarPV/Current Controller/Supply Current to dq/90 degree Phase shift ==
  In : Inport
  Gain : Gain  Gain=2
  Transfer Fcn : TransferFcn  Denominator=[1/(2*pi*grid.frequency) 1]
  Transfer Fcn1 : TransferFcn  Denominator=[1/(2*pi*grid.frequency) 1]
  Out : Outport  VectorParamsAs1DForOutWhenUnconnected=off
  wires:
  Transfer Fcn1/1 -> Gain/1
  Gain/1 -> Out/1
  Transfer Fcn/1 -> Transfer Fcn1/1
  In/1 -> Transfer Fcn/1

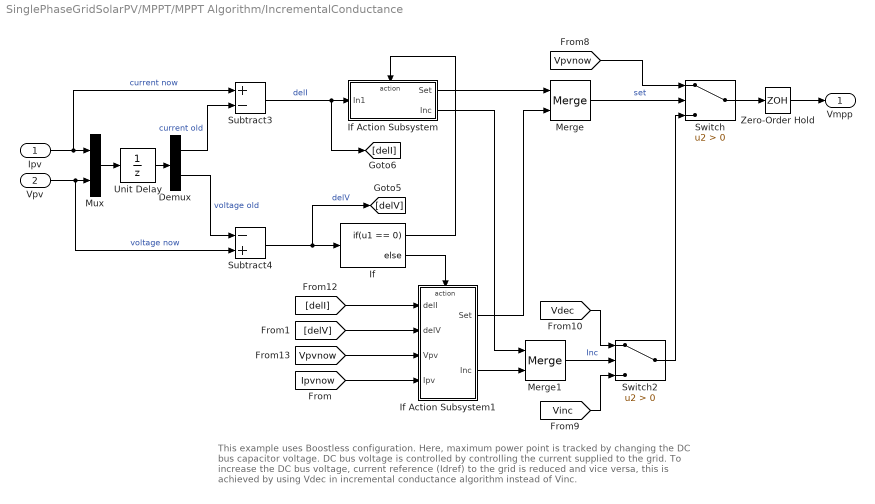
== system SinglePhaseGridSolarPV/MPPT/MPPT Algorithm/IncrementalConductance ==
  note: This example uses Boostless configuration. Here,  maximum power point is tracked by changing the DC bus capacitor voltage. DC bus voltage is controlled by controlling the current supplied to the grid.  To increase the DC bus voltage, current reference (Idref) to the grid is reduced and vice versa,
      | this is achieved by using Vdec in incremental conductance algorithm instead of Vinc.
  Ipv : Inport
  Vpv : Inport  Port=2
  Demux : Demux  Outputs=2
  If : If  IfExpression=u1 == 0
  If Action Subsystem : Subsystem  TreatAsAtomicUnit=on
  If Action Subsystem1 : Subsystem  TreatAsAtomicUnit=on
  Merge : Merge
  Merge1 : Merge
  Mux : Mux  Inputs=2
  Subtract3 : Sum  Inputs=+-
  Subtract4 : Sum  Inputs=-+
  Switch : Switch  Criteria=u2 > Threshold  SaturateOnIntegerOverflow=off  InputSameDT=off
  Switch2 : Switch  Criteria=u2 > Threshold  SaturateOnIntegerOverflow=off  InputSameDT=off
  Unit Delay : UnitDelay  InitialCondition=solarPlant.startMPPTValue  SampleTime=solarPlant.timeMPPT  HasFrameUpgradeWarning=on
  Zero-Order Hold : ZeroOrderHold  SampleTime=solarPlant.timeMPPT
  Vmpp : Outport  VectorParamsAs1DForOutWhenUnconnected=off
  wires:
  Merge1/1 -> Switch2/2  "Inc"
  [Vpvnow] -> Switch/1
  If Action Subsystem1/2(Inc) -> Merge1/2
  If Action Subsystem/2(Inc) -> Merge1/1
  If/2 -> If Action Subsystem1/Action
  If Action Subsystem/1(Set) -> Merge/1
  [delV] -> If Action Subsystem1/2(delV)
  [delI] -> If Action Subsystem1/1(delI)
  Merge/1 -> Switch/2  "set"
  If Action Subsystem1/1(Set) -> Merge/2
  If/1 -> If Action Subsystem/Action
  [Vpvnow] -> If Action Subsystem1/3(Vpv)
  Switch2/1 -> Switch/3
  [Ipvnow] -> If Action Subsystem1/4(Ipv)
  Ipv/1 -> Mux/1, Subtract3/1  "current now"
  Unit Delay/1 -> Demux/1
  Mux/1 -> Unit Delay/1
  Vpv/1 -> Subtract4/2, Mux/2  "voltage now"
  Demux/2 -> Subtract4/1  "voltage old"
  Demux/1 -> Subtract3/2  "current old"
  Subtract3/1 -> [delI], If Action Subsystem/1(In1)  "delI"
  Subtract4/1 -> [delV], If/1  "delV"
  [Vdec] -> Switch2/1
  [Vinc] -> Switch2/3
  Switch/1 -> Zero-Order Hold/1
  Zero-Order Hold/1 -> Vmpp/1

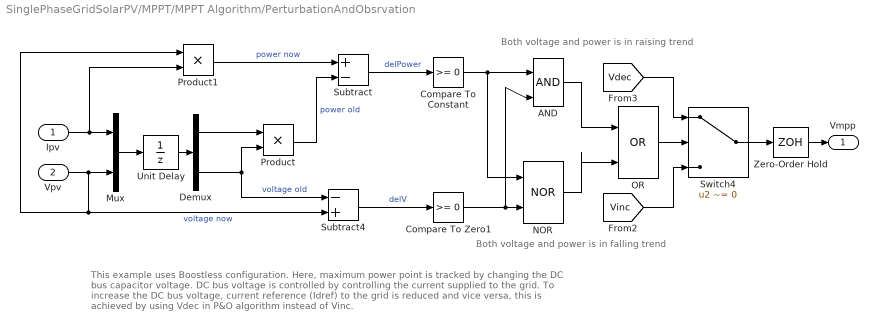
== system SinglePhaseGridSolarPV/MPPT/MPPT Algorithm/PerturbationAndObsrvation ==
  note: Both voltage and power is in falling trend
  note: Both voltage and power is in raising trend
  note: This example uses Boostless configuration. Here,  maximum power point is tracked by changing the DC bus capacitor voltage. DC bus voltage is controlled by controlling the current supplied to the grid.  To increase the DC bus voltage, current reference (Idref) to the grid is reduced and vice versa,
      | this is achieved by using Vdec in P&O algorithm instead of Vinc.
  Ipv : Inport
  Vpv : Inport  Port=2
  AND : Logic  IconShape=distinctive  AllPortsSameDT=off  OutDataTypeStr=boolean
  Compare To Constant : simulink/Logic and Bit Operations/Compare To Constant  relop=>=  const=0  OutDataTypeStr=boolean
  Compare To Zero1 : simulink/Logic and Bit Operations/Compare To Zero  relop=>=  OutDataTypeStr=boolean
  Demux : Demux  Outputs=2
  Mux : Mux  Inputs=2
  NOR : Logic  Operator=NOR  IconShape=distinctive  AllPortsSameDT=off  OutDataTypeStr=boolean
  OR : Logic  Operator=OR  IconShape=distinctive  AllPortsSameDT=off  OutDataTypeStr=boolean
  Product : Product
  Product1 : Product
  Subtract : Sum  Inputs=+-
  Subtract4 : Sum  Inputs=-+
  Switch4 : Switch  Criteria=u2 ~= 0  SaturateOnIntegerOverflow=off  InputSameDT=off
  Unit Delay : UnitDelay  InitialCondition=solarPlant.startMPPTValue  SampleTime=solarPlant.timeMPPT  HasFrameUpgradeWarning=on
  Zero-Order Hold : ZeroOrderHold  SampleTime=solarPlant.timeMPPT
  Vmpp : Outport  VectorParamsAs1DForOutWhenUnconnected=off
  wires:
  NOR/1 -> OR/2
  OR/1 -> Switch4/2
  Compare To Zero1/1 -> AND/2, NOR/2
  AND/1 -> OR/1
  Compare To Constant/1 -> AND/1, NOR/1
  Mux/1 -> Unit Delay/1
  Ipv/1 -> Product1/2, Mux/1
  Demux/1 -> Product/1
  Unit Delay/1 -> Demux/1
  Demux/2 -> Product/2, Subtract4/1  "voltage old"
  Vpv/1 -> Subtract4/2, Product1/1, Mux/2  "voltage now"
  Product1/1 -> Subtract/1  "power now"
  Product/1 -> Subtract/2  "power old"
  Subtract4/1 -> Compare To Zero1/1  "delV"
  Subtract/1 -> Compare To Constant/1  "delPower"
  Switch4/1 -> Zero-Order Hold/1
  Zero-Order Hold/1 -> Vmpp/1
  [Vinc] -> Switch4/3
  [Vdec] -> Switch4/1

== system SinglePhaseGridSolarPV/PLL and Protection/Protection/DC Bus Voltage ==
  Vpv : Inport
  Compare To Constant5 : simulink/Logic and Bit Operations/Compare To Constant  relop=>  const=protection.dcBusVoltageTripTime  OutDataTypeStr=boolean
  Compare To Constant6 : simulink/Logic and Bit Operations/Compare To Constant  relop=>  const=protection.dcBusMaxVoltage  OutDataTypeStr=boolean
  Compare To Constant7 : simulink/Logic and Bit Operations/Compare To Constant  relop=<  const=protection.dcBusMinVoltage  OutDataTypeStr=boolean
  Data Type Conversion1 : DataTypeConversion  SaturateOnIntegerOverflow=off  RndMeth=Floor
  Integrator1 : Integrator  ExternalReset=falling
  OR2 : Logic  Operator=OR  IconShape=distinctive  AllPortsSameDT=off  OutDataTypeStr=boolean
  Transfer Fcn2 : TransferFcn  Denominator=[1e-4 1]
  TripSig : Outport  VectorParamsAs1DForOutWhenUnconnected=off
  wires:
  Compare To Constant6/1 -> OR2/2
  Transfer Fcn2/1 -> Compare To Constant6/1, Compare To Constant7/1
  Compare To Constant7/1 -> OR2/1
  Vpv/1 -> Transfer Fcn2/1
  Integrator1/1 -> Compare To Constant5/1
  Data Type Conversion1/1 -> Integrator1/2, Integrator1/1
  OR2/1 -> Data Type Conversion1/1
  Compare To Constant5/1 -> TripSig/1

== system SinglePhaseGridSolarPV/PLL and Protection/Protection/Enabled Subsystem ==
  In : Inport
  Enable : EnablePort
  TripSig : Outport  InitialOutput=0  VectorParamsAs1DForOutWhenUnconnected=off
  wires:
  In/1 -> TripSig/1

== system SinglePhaseGridSolarPV/PLL and Protection/Protection/Grid Frequency ==
  w : Inport
  Compare To Constant2 : simulink/Logic and Bit Operations/Compare To Constant  relop=>  const=protection.gridMaxFreq*2*pi  OutDataTypeStr=boolean
  Compare To Constant3 : simulink/Logic and Bit Operations/Compare To Constant  relop=<  const=protection.gridMinFreq*2*pi  OutDataTypeStr=boolean
  Compare To Constant5 : simulink/Logic and Bit Operations/Compare To Constant  relop=>  const=protection.gridFrequencyTripTime  OutDataTypeStr=boolean
  Data Type Conversion1 : DataTypeConversion  SaturateOnIntegerOverflow=off  RndMeth=Floor
  Integrator1 : Integrator  ExternalReset=falling
  OR1 : Logic  Operator=OR  IconShape=distinctive  AllPortsSameDT=off  OutDataTypeStr=boolean
  Transfer Fcn1 : TransferFcn  Denominator=[1e-2 1]
  TripSig : Outport  VectorParamsAs1DForOutWhenUnconnected=off
  wires:
  Compare To Constant5/1 -> TripSig/1
  Transfer Fcn1/1 -> Compare To Constant2/1, Compare To Constant3/1
  Data Type Conversion1/1 -> Integrator1/2, Integrator1/1
  w/1 -> Transfer Fcn1/1
  Integrator1/1 -> Compare To Constant5/1
  OR1/1 -> Data Type Conversion1/1
  Compare To Constant2/1 -> OR1/1
  Compare To Constant3/1 -> OR1/2

== system SinglePhaseGridSolarPV/PLL and Protection/Protection/Grid Over Current ==
  Iac : Inport
  Compare To Constant8 : simulink/Logic and Bit Operations/Compare To Constant  relop=>  const=protection.overLoadCurrentTripTime  OutDataTypeStr=boolean
  Compare To Constant9 : simulink/Logic and Bit Operations/Compare To Constant  relop=>  const=protection.overLoadCurrent  OutDataTypeStr=boolean
  Data Type Conversion3 : DataTypeConversion  SaturateOnIntegerOverflow=off  RndMeth=Floor
  Integrator2 : Integrator  ExternalReset=falling
  RMS Measurement : eeRmsMeasurement/RMS Measurement  LabelModeActiveChoice=Total  F=grid.frequency  SpecifyHarmonics=off  K=[0 1 2]  Ts=1/(20*grid.frequency)
  TripSig : Outport  VectorParamsAs1DForOutWhenUnconnected=off
  wires:
  Compare To Constant9/1 -> Data Type Conversion3/1
  Data Type Conversion3/1 -> Integrator2/2, Integrator2/1
  Integrator2/1 -> Compare To Constant8/1
  Iac/1 -> RMS Measurement/1
  Compare To Constant8/1 -> TripSig/1
  RMS Measurement/1 -> Compare To Constant9/1

== system SinglePhaseGridSolarPV/PLL and Protection/Protection/Grid Voltage ==
  Vsd : Inport
  Compare To Constant : simulink/Logic and Bit Operations/Compare To Constant  relop=>  const=protection.gridMaxVoltage  OutDataTypeStr=boolean
  Compare To Constant1 : simulink/Logic and Bit Operations/Compare To Constant  relop=<  const=protection.gridMinVoltage  OutDataTypeStr=boolean
  Compare To Constant4 : simulink/Logic and Bit Operations/Compare To Constant  relop=>  const=protection.gridVoltageTripTime  OutDataTypeStr=boolean
  Data Type Conversion : DataTypeConversion  SaturateOnIntegerOverflow=off  RndMeth=Floor
  Integrator : Integrator  ExternalReset=falling
  OR : Logic  Operator=OR  IconShape=distinctive  AllPortsSameDT=off  OutDataTypeStr=boolean
  Transfer Fcn : TransferFcn  Denominator=[1e-3 1]
  Tripsig : Outport  VectorParamsAs1DForOutWhenUnconnected=off
  wires:
  OR/1 -> Data Type Conversion/1
  Data Type Conversion/1 -> Integrator/2, Integrator/1
  Transfer Fcn/1 -> Compare To Constant/1, Compare To Constant1/1
  Vsd/1 -> Transfer Fcn/1
  Integrator/1 -> Compare To Constant4/1
  Compare To Constant1/1 -> OR/1
  Compare To Constant/1 -> OR/2
  Compare To Constant4/1 -> Tripsig/1

== system SinglePhaseGridSolarPV/PLL and Protection/Protection/Short Circuit Current ==
  Iac : Inport
  AND : Logic  IconShape=distinctive  AllPortsSameDT=off  OutDataTypeStr=boolean
  Abs : Abs  SaturateOnIntegerOverflow=off
  Clock : Clock
  Compare To Constant : simulink/Logic and Bit Operations/Compare To Constant  relop=>  const=protection.shortCircuitCurrentStartTime  OutDataTypeStr=boolean
  Compare To Constant11 : simulink/Logic and Bit Operations/Compare To Constant  relop=>  const=protection.shortCircuitCurrent  OutDataTypeStr=boolean
  TripSig : Outport  VectorParamsAs1DForOutWhenUnconnected=off
  wires:
  Compare To Constant11/1 -> AND/1
  Iac/1 -> Abs/1
  Abs/1 -> Compare To Constant11/1
  Clock/1 -> Compare To Constant/1
  Compare To Constant/1 -> AND/2
  AND/1 -> TripSig/1

== system SinglePhaseGridSolarPV/Power Circuit/Power Circuit/Average ==
  m : Inport
  TripSig : Inport  Port=2
  Average-Value Chopper : ee_lib/Semiconductors & Converters/Converters/Average-Value Chopper  chopper_type=5  efficiency_option=1  efficiency_fixed=100  i_vec=[0, 2, 5] A  efficiency_vec=[90, 95, 98]
      settings: InternalSimscapePortConfiguration="{\"Bottom\":[],\"Left\":[{\"id\":\"DutyCycle\",\"label\":\"DutyCycle\",\"type\":\"input\"},{\"id\":\"p1\",\"label\":\"1+\",\"type\":\"foundation.electrical.electrical\"},{\"id\":\"n1\",\"label\":\"1-\",\"type\":\"foundation.electrical.electrical\"}],\"Right\":[{\"id\":\"p2\",\"label\":\"2+\",\"type\":\"foundation.electrical.electrical\"},{\"id\":\"n2\",\"label\":\"2-\",\"type\":\"foundation.electrical.electrical\"}],\"Top\":[]}"
  Map [-1,1] to [0,1] : Subsystem
  Simulink-PS Converter2 : nesl_utility/Simulink-PS Converter  PhysicalDomain=network_engine_domain  SubClassName=ps_input  LeftPortType=input  RightPortType=output  PseudoPeriodic=off  Frequencies=[]  NoiseDistribution=none  NoiseParameters=[]  Unit=1  AffineConversion=off  FilteringAndDerivatives=provide  SimscapeFilterOrder=1  InputFilterTimeConstant=0.001  UdotUserProvided=0
  Terminator : Terminator
  P : PMIOPort  Side=Right
  + : PMIOPort  Port=2  Side=Left
  - : PMIOPort  Port=3  Side=Left
  N : PMIOPort  Port=4  Side=Right
  wires:
  m/1 -> Simulink-PS Converter2/1
  TripSig/1 -> Terminator/1
  connections:
  Simulink-PS Converter2/RConn1 -- Map [-1,1] to [0,1]/LConn1
  Map [-1,1] to [0,1]/RConn1 -- Average-Value Chopper/LConn1
  P/RConn1 -- Average-Value Chopper/RConn1
  N/RConn1 -- Average-Value Chopper/RConn2
  Average-Value Chopper/LConn3 -- -/RConn1
  +/RConn1 -- Average-Value Chopper/LConn2
